simulink subsystem "Controller3w"  (R2025b)
settings: Solver=VariableStepAuto  StartTime=0.0  StopTime=10.0  RelTol=1e-3
undefined symbols (not defined in the file or in its folder): battery, controller, drivetrain
libraries: BatteryCurrentManagement x2
settings Model: Creator=jjha  LastModifiedBy=jjha
settings OptimizationCC: ReuseModelBlockBuffer=off
settings RTWCC: GPUComputeCapability=3.5

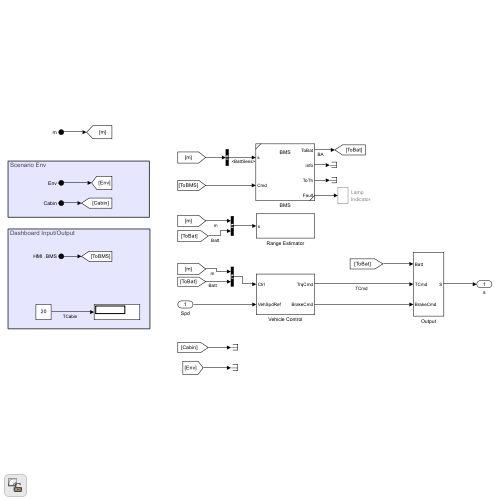
[thumbnail: Simulink's stored preview of the top-level diagram]
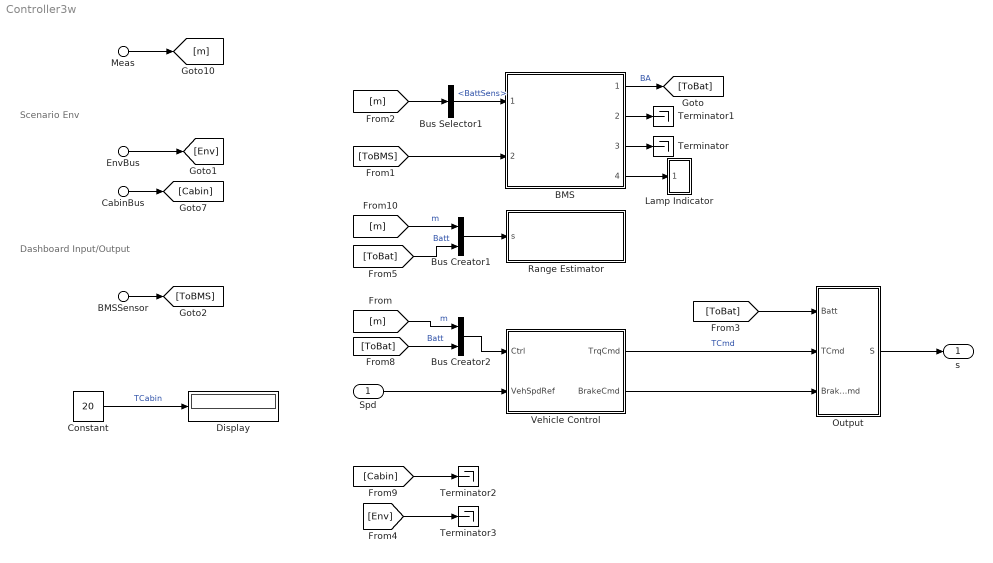
== system Controller3w ==
  note: Scenario Env
  note: Dashboard Input/Output
  Spd : Inport
  EnvBus : Inport  Port=2  PortName=Env
  CabinBus : Inport  Port=3  PortName=Cabin
  Meas : Inport  Port=4  PortName=m
  BMSSensor : Inport  Port=5  PortName=HMI  Element=BMS
  BMS : Subsystem  ReferencedSubsystem=BMS
      settings: PortSchema="{\"entries\":[{\"content\":{\"sides\":[{\"content\":{},\"type\":\"ConnectorPlacement.EquallySpacedRectSide\",\"uuid\":\"92c05094-f9b0-45a3-ac1b-1858c0c996e8\"},{\"content\":{\"side\":\"RIGHT\"},\"type\":\"ConnectorPlacement.EquallySpacedRectSide\",\"uuid\":\"cdc13757-7d0c-4e35-a976-de64c06d8cde\"},{\"content\":{\"connectorIds\":[\"In1\",\"In2\"],\"side\":\"TOP\"},\"type\":\"ConnectorPlacement.EquallySpacedRectSide\",\"uuid\":\"c53a1ad0-a5f6-468e-b5dd-f0a27cee9942\"},{\"content\":{\"connectorIds\":[\"Out1\",\"Out2\",\"Out3\",\"Out4\"],\"side\":\"BOTTOM\"},\"type\":\"ConnectorPlacement.EquallySpacedRectSide\",\"uuid\":\"8abfd502-0389-4393-bb18-f131709acb23\"}]},\"type\":\"ConnectorPlacement.EquallySpacedConnector\",\"uuid\":\"102d552e-f167-4796-a536-13938ac07fac\"}],\"packageUris\":[\"http://schema.mathworks.com/mf0/Connector/R2020b\"],\"version\":\"1.0\"}"
  Bus Creator1 : BusCreator  Inputs=2
  Bus Creator2 : BusCreator  Inputs=2
  Bus Selector1 : BusSelector  OutputSignals=BA.BattSens
  Constant : Constant  Value=20
  Display : Display
  Lamp Indicator : Subsystem
      settings: PortSchema="{\"entries\":[{\"content\":{\"sides\":[{\"content\":{\"connectorIds\":[]},\"type\":\"ConnectorPlacement.EquallySpacedRectSide\",\"uuid\":\"c55e4a0c-c727-4224-8aa6-2961c151763f\"},{\"content\":{\"connectorIds\":[],\"side\":\"RIGHT\"},\"type\":\"ConnectorPlacement.EquallySpacedRectSide\",\"uuid\":\"62aa4b95-0b95-454c-8041-b3e5f6582f45\"},{\"content\":{\"connectorIds\":[\"In1\"],\"side\":\"TOP\"},\"type\":\"ConnectorPlacement.EquallySpacedRectSide\",\"uuid\":\"0d235e8c-306c-4ade-b7e4-bd2fcf6610c8\"}]},\"type\":\"ConnectorPlacement.EquallySpacedConnector\",\"uuid\":\"6725a8d5-e875-410a-8026-694fde1b795b\"}],\"packageUris\":[\"http://schema.mathworks.com/mf0/Connector/R2020b\"],\"version\":\"1.0\"}"
  Output : Subsystem
  Range Estimator : Subsystem
  Terminator{,1..3} (4 alike) : Terminator
  Vehicle Control : Subsystem
  s : Outport
  wires:
  [ToBat] -> Bus Creator1/2  "Batt"
  Bus Selector1/1 -> BMS/1  "<BattSens>"
  BMS/2 -> Terminator1/1
  BMS/4 -> Lamp Indicator/1(" ")
  BMS/3 -> Terminator/1
  BMS/1 -> [ToBat]  "BA"
  Spd/1 -> Vehicle Control/2(VehSpdRef)
  Meas/1 -> [m]
  EnvBus/1 -> [Env]
  CabinBus/1 -> [Cabin]
  Bus Creator1/1 -> Range Estimator/1(s)
  [ToBat] -> Bus Creator2/2  "Batt"
  Bus Creator2/1 -> Vehicle Control/1(Ctrl)
  [m] -> Bus Creator2/1  "m"
  [m] -> Bus Selector1/1
  [m] -> Bus Creator1/1  "m"
  [ToBMS] -> BMS/2
  BMSSensor/1 -> [ToBMS]
  [Cabin] -> Terminator2/1
  Constant/1 -> Display/1  "TCabin"
  [Env] -> Terminator3/1
  Vehicle Control/2(BrakeCmd) -> Output/3(BrakeCmd)
  [ToBat] -> Output/1(Batt)
  Output/1(S) -> s/1
  Vehicle Control/1(TrqCmd) -> Output/2(TCmd)  "TCmd"

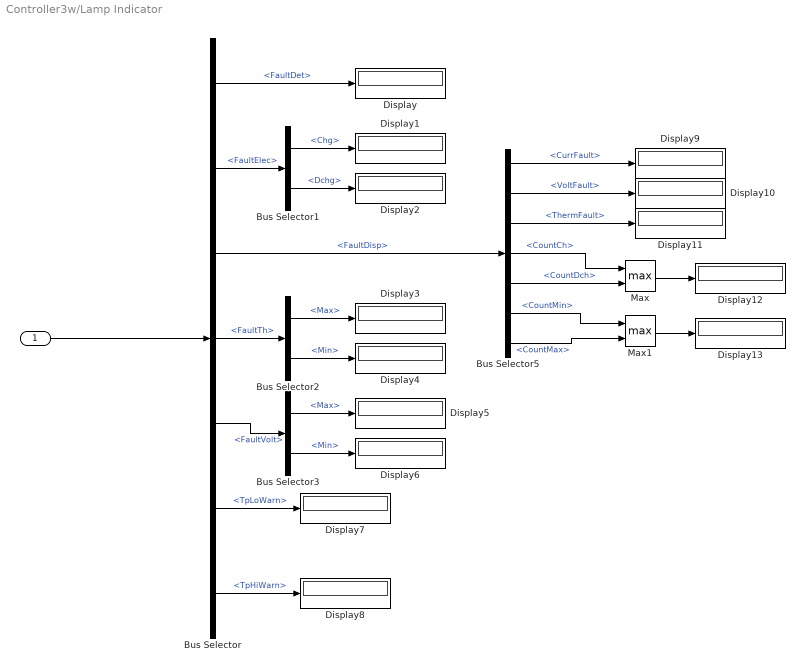
== system Controller3w/Lamp Indicator ==
  " " : Inport
  Bus Selector : BusSelector  OutputSignals=Fault.FaultDet,Fault.FaultElec,Fault.FaultDisp,Fault.FaultTh,Fault.FaultVolt,TpLoWarn,TpHiWarn
  Bus Selector1 : BusSelector  OutputSignals=Chg,Dchg
  Bus Selector2 : BusSelector  OutputSignals=Max,Min
  Bus Selector3 : BusSelector  OutputSignals=Max,Min
  Bus Selector5 : BusSelector  OutputSignals=CurrFault,VoltFault,ThermFault,CountCh,CountDch,CountMin,CountMax
  Display{,1..13} (14 alike) : Display
  Max : MinMax  Function=max  Inputs=2
  Max1 : MinMax  Function=max  Inputs=2
  wires:
  " "/1 -> Bus Selector/1
  Bus Selector/1 -> Display/1  "<FaultDet>"
  Bus Selector/2 -> Bus Selector1/1  "<FaultElec>"
  Bus Selector1/1 -> Display1/1  "<Chg>"
  Bus Selector1/2 -> Display2/1  "<Dchg>"
  Bus Selector/4 -> Bus Selector2/1  "<FaultTh>"
  Bus Selector2/2 -> Display4/1  "<Min>"
  Bus Selector2/1 -> Display3/1  "<Max>"
  Bus Selector3/1 -> Display5/1  "<Max>"
  Bus Selector3/2 -> Display6/1  "<Min>"
  Bus Selector/5 -> Bus Selector3/1  "<FaultVolt>"
  Bus Selector/6 -> Display7/1  "<TpLoWarn>"
  Bus Selector/7 -> Display8/1  "<TpHiWarn>"
  Bus Selector/3 -> Bus Selector5/1  "<FaultDisp>"
  Bus Selector5/1 -> Display9/1  "<CurrFault>"
  Bus Selector5/2 -> Display10/1  "<VoltFault>"
  Bus Selector5/3 -> Display11/1  "<ThermFault>"
  Bus Selector5/4 -> Max/1  "<CountCh>"
  Bus Selector5/6 -> Max1/1  "<CountMin>"
  Bus Selector5/7 -> Max1/2  "<CountMax>"
  Bus Selector5/5 -> Max/2  "<CountDch>"
  Max/1 -> Display12/1
  Max1/1 -> Display13/1

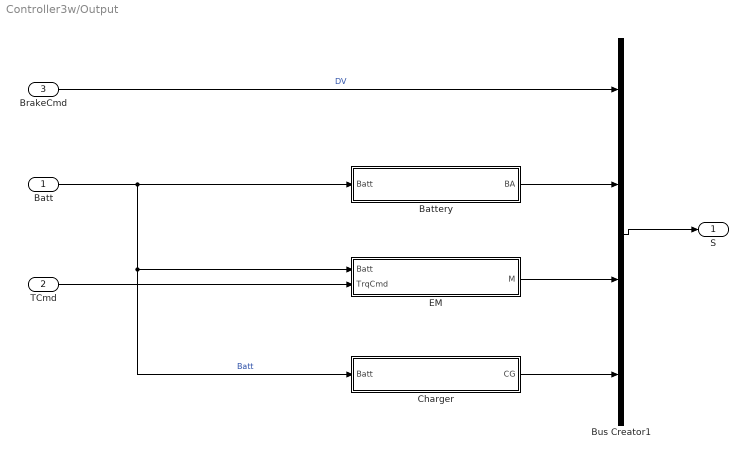
== system Controller3w/Output ==
  Batt : Inport
  TCmd : Inport  Port=2
  BrakeCmd : Inport  Port=3
  Battery : Subsystem
      mask Display: disp(get_param(gcb, 'Name'))
  Bus Creator1 : BusCreator  Inputs=4
  Charger : Subsystem
      mask Display: disp(get_param(gcb, 'Name'))
  EM : Subsystem
      mask Display: disp(get_param(gcb, 'Name'))
  S : Outport
  wires:
  Bus Creator1/1 -> S/1
  TCmd/1 -> EM/2(TrqCmd)
  EM/1(M) -> Bus Creator1/3
  Battery/1(BA) -> Bus Creator1/2
  Batt/1 -> Battery/1(Batt), EM/1(Batt), Charger/1(Batt)  "Batt"
  Charger/1(CG) -> Bus Creator1/4
  BrakeCmd/1 -> Bus Creator1/1  "DV"

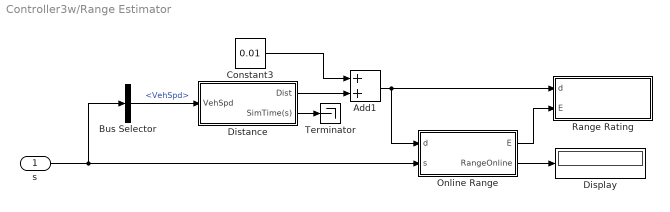
== system Controller3w/Range Estimator ==
  s : Inport
  Add1 : Sum
  Bus Selector : BusSelector  OutputSignals=m.DV.VehSpd
  Constant3 : Constant  Value=0.01
  Display : Display
  Distance : Subsystem
  Online Range : Subsystem
  Range Rating : Subsystem
  Terminator : Terminator
  wires:
  Online Range/1(E) -> Range Rating/2(E)
  Online Range/2(RangeOnline) -> Display/1
  s/1 -> Online Range/2(s), Bus Selector/1
  Constant3/1 -> Add1/1
  Bus Selector/1 -> Distance/1(VehSpd)  "<VehSpd>"
  Distance/2(SimTime(s)) -> Terminator/1
  Add1/1 -> Range Rating/1(d), Online Range/1(d)
  Distance/1(Dist) -> Add1/2

== system Controller3w/Vehicle Control ==
  Ctrl : Inport
  VehSpdRef : Inport  Port=2
  Bus Selector : BusSelector  OutputSignals=m.M.EM.EMrpm
  Driver : Subsystem
  Torque Control : Subsystem
  Torque Req : Subsystem
  TrqCmd : Outport
  BrakeCmd : Outport  Port=2
  wires:
  VehSpdRef/1 -> Driver/1(VehSpdRef)
  Bus Selector/1 -> Driver/2(rpm)  "<EMrpm>"
  Driver/1(TrqReq) -> Torque Control/1(TrqReq)
  Ctrl/1 -> Bus Selector/1, Torque Control/2(Crtl)
  Torque Req/1(TrqCmd) -> TrqCmd/1
  Torque Control/1(TrqCtrl) -> Torque Req/1(TrqCtrl)
  Torque Req/2(BrakeCmd) -> BrakeCmd/1

== system Controller3w/Output/Battery ==
  Batt : Inport
  Bus Creator : BusCreator  Inputs=2
  Bus Selector : BusSelector  OutputSignals=Relay.RelayPos,Relay.RelayNeg
  BA : Outport
  wires:
  Bus Selector/1 -> Bus Creator/1  "<RelayPos>"
  Batt/1 -> Bus Selector/1  "BA"
  Bus Selector/2 -> Bus Creator/2  "<RelayNeg>"
  Bus Creator/1 -> BA/1  "BA"

== system Controller3w/Output/Charger ==
  Batt : Inport
  Bus Creator : BusCreator  Inputs=1
  CG : Outport
  wires:
  Bus Creator/1 -> CG/1  "CG"
  Batt/1 -> Bus Creator/1  "Batt"

== system Controller3w/Output/EM ==
  Batt : Inport
  TrqCmd : Inport  Port=2
  Bus Creator3 : BusCreator  Inputs=2
  Bus Selector1 : BusSelector  OutputSignals=TorqueCmd
  Gain : Gain
  Scope : Scope
  M : Outport
  wires:
  Gain/1 -> Bus Creator3/1, Scope/1  "EMtrq"
  Batt/1 -> Bus Creator3/2
  Bus Creator3/1 -> M/1  "M"
  Bus Selector1/1 -> Gain/1  "<TorqueCmd>"
  TrqCmd/1 -> Bus Selector1/1

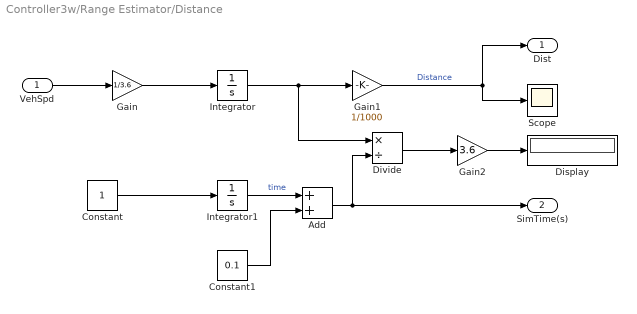
== system Controller3w/Range Estimator/Distance ==
  VehSpd : Inport
  Add : Sum
  Constant : Constant
  Constant1 : Constant  Value=0.1
  Display : Display
  Divide : Product  Inputs=*/
  Gain : Gain  Gain=1/3.6
  Gain1 : Gain  Gain=1/1000
  Gain2 : Gain  Gain=3.6
  Integrator : Integrator
  Integrator1 : Integrator
  Scope : Scope
      settings: ActiveDisplayYMinimum=-40.29184  ActiveDisplayYMaximum=362.62657  DataLoggingVariableName=ScopeData2
  Dist : Outport
  SimTime(s) : Outport  Port=2
  wires:
  Gain2/1 -> Display/1
  Gain1/1 -> Dist/1, Scope/1  "Distance"
  Gain/1 -> Integrator/1
  Divide/1 -> Gain2/1
  Add/1 -> SimTime(s)/1, Divide/2
  Integrator1/1 -> Add/1  "time"
  Constant1/1 -> Add/2
  Integrator/1 -> Divide/1, Gain1/1
  VehSpd/1 -> Gain/1
  Constant/1 -> Integrator1/1

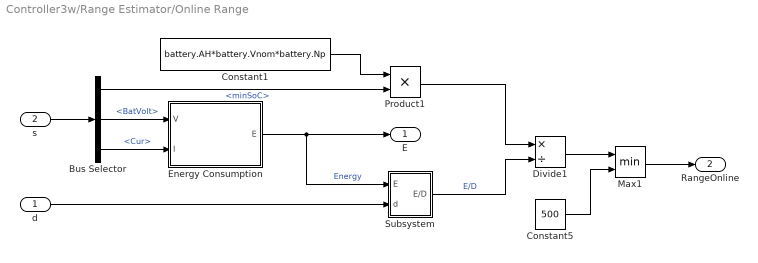
== system Controller3w/Range Estimator/Online Range ==
  d : Inport
  s : Inport  Port=2
  Bus Selector : BusSelector  OutputSignals=Batt.BattSensor.minSoC,Batt.BattSensor.BatVolt,Batt.BattSensor.Cur
  Constant1 : Constant  Value=battery.AH*battery.Vnom*battery.Np
  Constant5 : Constant  Value=500
  Divide1 : Product  Inputs=*/
  Energy Consumption : Subsystem
  Max1 : MinMax  Inputs=2  ZeroCross=off
  Product1 : Product
  Subsystem : Subsystem
  E : Outport
  RangeOnline : Outport  Port=2
  wires:
  Subsystem/1(E/D) -> Divide1/2  "E/D"
  d/1 -> Subsystem/2(d)
  Product1/1 -> Divide1/1
  Constant1/1 -> Product1/1
  Bus Selector/3 -> Energy Consumption/2(I)  "<Cur>"
  Bus Selector/2 -> Energy Consumption/1(V)  "<BatVolt>"
  Energy Consumption/1(E) -> E/1, Subsystem/1(E)  "Energy"
  s/1 -> Bus Selector/1
  Max1/1 -> RangeOnline/1
  Divide1/1 -> Max1/1
  Constant5/1 -> Max1/2
  Bus Selector/1 -> Product1/2  "<minSoC>"

== system Controller3w/Range Estimator/Range Rating ==
  note: Total capacity at full charge , Ahr*BatVoltage*CellinSeries
  d : Inport
  E : Inport  Port=2
  Add : Sum
  Constant : Constant
  Display : Display
  Divide : Product  Inputs=*/
  Divide1 : Product  Inputs=/*
  TotalEnergy : Constant  Value=battery.AH*battery.Vnom*battery.Np
  wires:
  Divide/1 -> Add/2
  Divide1/1 -> Display/1  "RangeRating"
  d/1 -> Divide/2
  E/1 -> Divide/1
  Constant/1 -> Add/1
  Add/1 -> Divide1/1
  TotalEnergy/1 -> Divide1/2

== system Controller3w/Vehicle Control/Driver ==
  VehSpdRef : Inport
  rpm : Inport  Port=2
  Motor Speed Reference : Subsystem
  Speed Controller : Subsystem
      settings: PortSchema="{\"entries\":[{\"content\":{\"sides\":[{\"content\":{\"connectorIds\":[\"Out1\"]},\"type\":\"ConnectorPlacement.EquallySpacedRectSide\",\"uuid\":\"12b9f2c9-2b28-451b-ad36-7fe4150db485\"},{\"content\":{\"connectorIds\":[\"In2\"],\"side\":\"RIGHT\"},\"type\":\"ConnectorPlacement.EquallySpacedRectSide\",\"uuid\":\"c0fdf9a4-483a-4ddc-b663-6299fcc79327\"},{\"content\":{\"connectorIds\":[\"In1\"],\"side\":\"TOP\"},\"type\":\"ConnectorPlacement.EquallySpacedRectSide\",\"uuid\":\"3f20082e-8487-45e3-9fd7-d6d75741df4d\"}]},\"type\":\"ConnectorPlacement.EquallySpacedConnector\",\"uuid\":\"9361cdd3-74d8-46ee-ae7f-e2dde5d31ed1\"}],\"packageUris\":[\"http://schema.mathworks.com/mf0/Connector/19700101\"],\"version\":\"1.0\"}"
  TrqReq : Outport
  wires:
  VehSpdRef/1 -> Motor Speed Reference/1(VehSpd)
  Speed Controller/1(TrqPID) -> TrqReq/1
  rpm/1 -> Speed Controller/1(Spd)
  Motor Speed Reference/1(MotorSpdRef) -> Speed Controller/2(SpdRef)

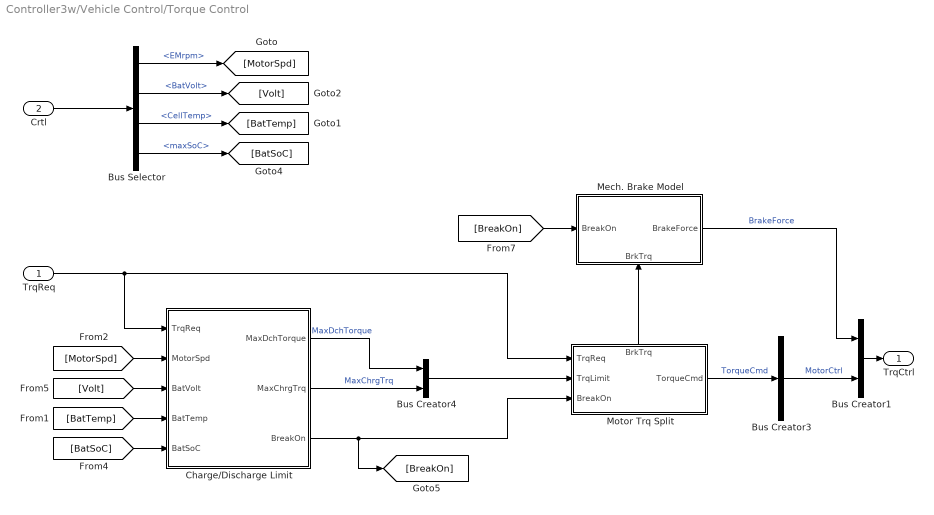
== system Controller3w/Vehicle Control/Torque Control ==
  TrqReq : Inport
  Crtl : Inport  Port=2
  Bus Creator1 : BusCreator  Inputs=2
  Bus Creator3 : BusCreator  Inputs=1
  Bus Creator4 : BusCreator  Inputs=2
  Bus Selector : BusSelector  OutputSignals=m.M.EM.EMrpm,Batt.BattSensor.BatVolt,Batt.BattSensor.CellTemp,Batt.BattSensor.maxSoC
  Charge/Discharge Limit : Subsystem
  Mech. Brake Model : Subsystem
      settings: PortSchema="{\"entries\":[{\"content\":{\"sides\":[{\"content\":{\"connectorIds\":[\"In1\"]},\"type\":\"ConnectorPlacement.EquallySpacedRectSide\",\"uuid\":\"3fcf8e06-a346-49b8-a4a8-b41cf2b27013\"},{\"content\":{\"connectorIds\":[\"Out1\"],\"side\":\"RIGHT\"},\"type\":\"ConnectorPlacement.EquallySpacedRectSide\",\"uuid\":\"8698242e-d004-4fda-889c-69f0784e7402\"},{\"content\":{\"connectorIds\":[],\"side\":\"TOP\"},\"type\":\"ConnectorPlacement.EquallySpacedRectSide\",\"uuid\":\"7829013b-7288-42bb-bccf-7e6edbe20d12\"},{\"content\":{\"connectorIds\":[\"In2\"],\"side\":\"BOTTOM\"},\"type\":\"ConnectorPlacement.EquallySpacedRectSide\",\"uuid\":\"357a4631-0a09-454f-b0f2-2b693ca62a9f\"},{\"content\":{\"connectorIds\":[],\"side\":\"HIDDEN\"},\"type\":\"ConnectorPlacement.EquallySpacedRectSide\",\"uuid\":\"b5eacf60-b578-4936-bef0-d59a279d5824\"}]},\"type\":\"ConnectorPlacement.EquallySpacedConnector\",\"uuid\":\"d2ebf12e-a3e7-4a55-b8c6-fa4e5ed13b89\"}],\"packageUris\":[\"http://schema.mathworks.com/mf0/Connector/R2020b\"],\"version\":\"1.0\"}"
  Motor Trq Split : Subsystem
      settings: PortSchema="{\"entries\":[{\"content\":{\"sides\":[{\"content\":{\"connectorIds\":[\"In1\",\"In2\",\"In3\"]},\"type\":\"ConnectorPlacement.EquallySpacedRectSide\",\"uuid\":\"c6883188-188e-4cbf-9dc5-1a26bf01b714\"},{\"content\":{\"connectorIds\":[\"Out1\"],\"side\":\"RIGHT\"},\"type\":\"ConnectorPlacement.EquallySpacedRectSide\",\"uuid\":\"b7c90991-838b-485d-9a4c-3fbacac28b54\"},{\"content\":{\"connectorIds\":[\"Out2\"],\"side\":\"TOP\"},\"type\":\"ConnectorPlacement.EquallySpacedRectSide\",\"uuid\":\"50e43671-3241-4bf5-a3b9-e23b27b7214a\"},{\"content\":{\"connectorIds\":[],\"side\":\"HIDDEN\"},\"type\":\"ConnectorPlacement.EquallySpacedRectSide\",\"uuid\":\"7c25a71e-e9cc-425c-8a3d-1b4aa412427f\"}]},\"type\":\"ConnectorPlacement.EquallySpacedConnector\",\"uuid\":\"d51dcaef-c892-4ef2-982d-c6c52760ceaa\"}],\"packageUris\":[\"http://schema.mathworks.com/mf0/Connector/R2020b\"],\"version\":\"1.0\"}"
  TrqCtrl : Outport
  wires:
  Crtl/1 -> Bus Selector/1
  Bus Selector/1 -> [MotorSpd]  "<EMrpm>"
  Bus Selector/4 -> [BatSoC]  "<maxSoC>"
  Bus Selector/2 -> [Volt]  "<BatVolt>"
  Bus Selector/3 -> [BatTemp]  "<CellTemp>"
  Charge/Discharge Limit/3(BreakOn) -> [BreakOn], Motor Trq Split/3(BreakOn)
  Charge/Discharge Limit/1(MaxDchTorque) -> Bus Creator4/1  "MaxDchTorque"
  TrqReq/1 -> Charge/Discharge Limit/1(TrqReq), Motor Trq Split/1(TrqReq)
  [MotorSpd] -> Charge/Discharge Limit/2(MotorSpd)
  [BatSoC] -> Charge/Discharge Limit/5(BatSoC)
  [BatTemp] -> Charge/Discharge Limit/4(BatTemp)
  [Volt] -> Charge/Discharge Limit/3(BatVolt)
  [BreakOn] -> Mech. Brake Model/1(BreakOn)
  Motor Trq Split/2(BrkTrq) -> Mech. Brake Model/2(BrkTrq)
  Charge/Discharge Limit/2(MaxChrgTrq) -> Bus Creator4/2  "MaxChrgTrq"
  Bus Creator4/1 -> Motor Trq Split/2(TrqLimit)
  Mech. Brake Model/1(BrakeForce) -> Bus Creator1/1  "BrakeForce"
  Bus Creator1/1 -> TrqCtrl/1
  Bus Creator3/1 -> Bus Creator1/2  "MotorCtrl"
  Motor Trq Split/1(TorqueCmd) -> Bus Creator3/1  "TorqueCmd"

== system Controller3w/Vehicle Control/Torque Req ==
  TrqCtrl : Inport
  Bus Selector1 : BusSelector  OutputSignals=BrakeForce,MotorCtrl.TorqueCmd
  TrqCmd : Outport
  BrakeCmd : Outport  Port=2
  wires:
  TrqCtrl/1 -> Bus Selector1/1
  Bus Selector1/2 -> TrqCmd/1  "<TorqueCmd>"
  Bus Selector1/1 -> BrakeCmd/1  "<BrakeForce>"

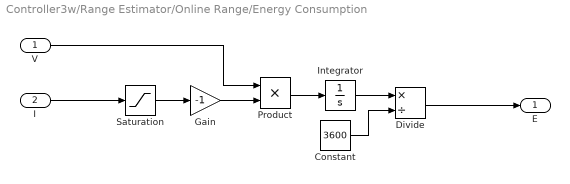
== system Controller3w/Range Estimator/Online Range/Energy Consumption ==
  V : Inport
  I : Inport  Port=2
  Constant : Constant  Value=3600
  Divide : Product  Inputs=*/
  Gain : Gain  Gain=-1
  Integrator : Integrator
  Product : Product
  Saturation : Saturate  UpperLimit=0  LowerLimit=-inf  ZeroCross=off
  E : Outport
  wires:
  Gain/1 -> Product/2
  Divide/1 -> E/1
  V/1 -> Product/1
  I/1 -> Saturation/1
  Product/1 -> Integrator/1
  Integrator/1 -> Divide/1
  Constant/1 -> Divide/2
  Saturation/1 -> Gain/1

== system Controller3w/Range Estimator/Online Range/Subsystem ==
  E : Inport
  d : Inport  Port=2
  Add : Sum
  Constant2 : Constant
  Divide2 : Product  Inputs=*/
  E/D : Outport
  wires:
  E/1 -> Divide2/1
  d/1 -> Divide2/2
  Divide2/1 -> Add/1
  Constant2/1 -> Add/2
  Add/1 -> E/D/1

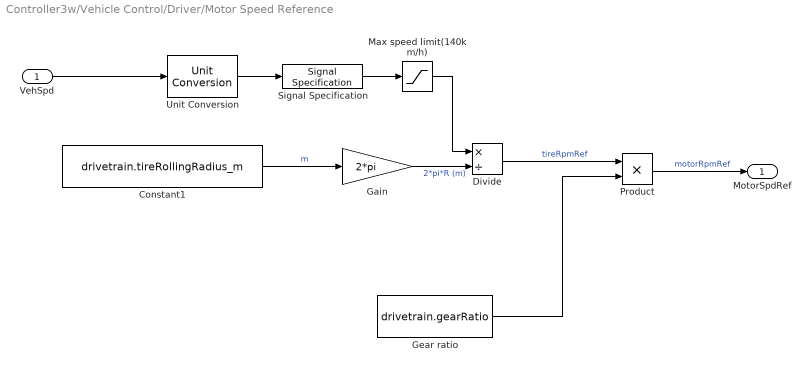
== system Controller3w/Vehicle Control/Driver/Motor Speed Reference ==
  VehSpd : Inport  Unit=km/hr
  Constant1 : Constant  Value=drivetrain.tireRollingRadius_m
  Divide : Product  Inputs=*/
  Gain : Gain  Gain=2*pi
  Gear ratio : Constant  Value=drivetrain.gearRatio
  Max speed limit(140km/h) : Saturate  UpperLimit=drivetrain.MaxSpeed  LowerLimit=0  ZeroCross=off
  Product : Product
  Signal Specification : SignalSpecification  Unit=m/min
  Unit Conversion : UnitConversion
  MotorSpdRef : Outport  Unit=rpm  VectorParamsAs1DForOutWhenUnconnected=off
  wires:
  Max speed limit(140km/h)/1 -> Divide/1
  VehSpd/1 -> Unit Conversion/1
  Product/1 -> MotorSpdRef/1  "motorRpmRef"
  Gear ratio/1 -> Product/2
  Divide/1 -> Product/1  "tireRpmRef"
  Gain/1 -> Divide/2  "2*pi*R (m)"
  Signal Specification/1 -> Max speed limit(140km/h)/1
  Unit Conversion/1 -> Signal Specification/1
  Constant1/1 -> Gain/1  "m"

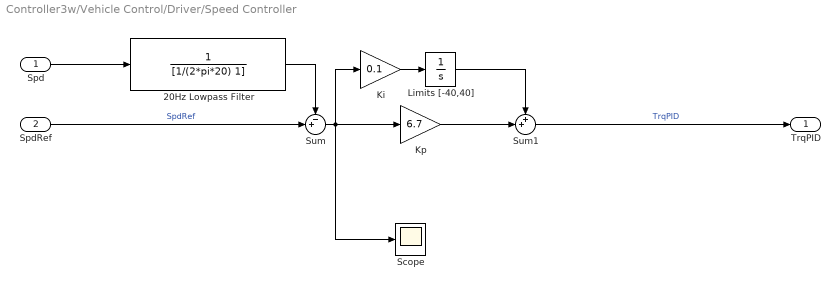
== system Controller3w/Vehicle Control/Driver/Speed Controller ==
  Spd : Inport  Unit=rpm
      settings: AttributesFormatString=%<Unit>
  SpdRef : Inport  Port=2  Unit=rpm
      settings: AttributesFormatString=%<Unit>
  20Hz Lowpass Filter : TransferFcn  Denominator=[1/(2*pi*20) 1]
  Ki : Gain  Gain=0.1
  Kp : Gain  Gain=6.7
  Limits [-40,40] : Integrator  LimitOutput=on  UpperSaturationLimit=40  LowerSaturationLimit=-40  ZeroCross=off
  Scope : Scope
      settings: ActiveDisplayYMinimum=-356.59933  ActiveDisplayYMaximum=2361.12393
  Sum : Sum  Inputs=-+|
  Sum1 : Sum  Inputs=++|
  TrqPID : Outport  Unit=N*m  VectorParamsAs1DForOutWhenUnconnected=off
      settings: AttributesFormatString=%<Unit>
  wires:
  SpdRef/1 -> Sum/2  "SpdRef"
  Spd/1 -> 20Hz Lowpass Filter/1
  Ki/1 -> Limits [-40,40]/1
  20Hz Lowpass Filter/1 -> Sum/1
  Sum/1 -> Ki/1, Kp/1, Scope/1
  Kp/1 -> Sum1/2
  Limits [-40,40]/1 -> Sum1/1
  Sum1/1 -> TrqPID/1  "TrqPID"

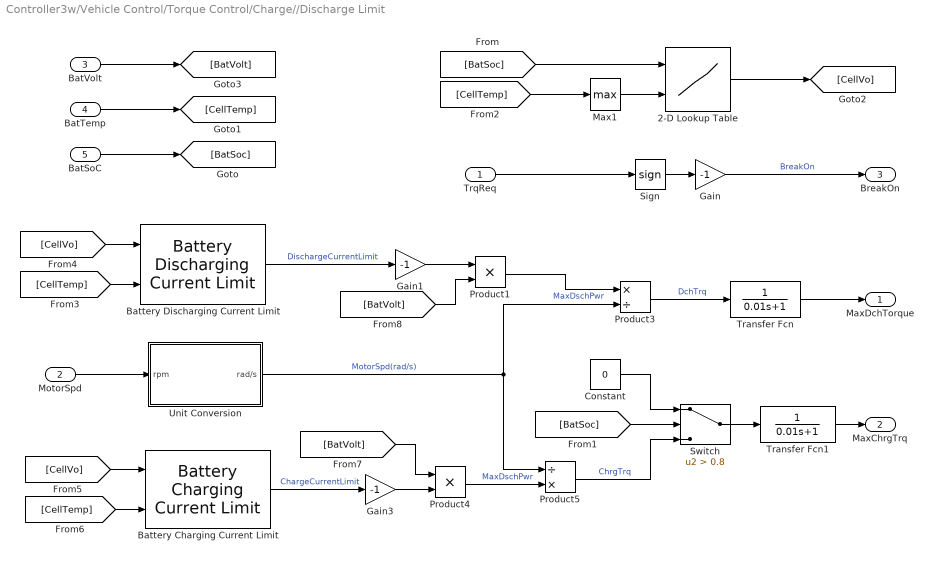
== system Controller3w/Vehicle Control/Torque Control/Charge//Discharge Limit ==
  TrqReq : Inport
  MotorSpd : Inport  Port=2
  BatVolt : Inport  Port=3
  BatTemp : Inport  Port=4
  BatSoC : Inport  Port=5
  2-D Lookup Table : Lookup_n-D  BreakpointsForDimension1=battery.SOC_vec  BreakpointsForDimension2=battery.T_vec  Table=battery.V0_mat  InternalRulePriority=Speed  RndMeth=Simplest
      settings: InputPortMap=u0,u1
  Battery Charging Current Limit : BatteryCurrentManagement/Battery Charging Current Limit  MinMaxFlag=off  CellOvervoltageLimit=4.5  R0=0.0025  T_vec=[243.15, 258.15, 273.15, 288.15, 303.15, 318.15, 333.15]  CurrentLimitCoolestCell=[ 0, 0,0.5* battery.AH, battery.AH, battery.AH, battery.AH, battery.AH]  CurrentLimitHottestCell="[ battery.AH,  battery.AH,  battery.AH,  battery.AH,  battery.AH,  0.5*battery.AH, 0]"  DataType=Inherit: auto
  Battery Discharging Current Limit : BatteryCurrentManagement/Battery Discharging Current Limit  MinMaxFlag=off  CellUndervoltageLimit=3  R0=0.0025  T_vec=[243.15, 258.15, 273.15, 288.15, 303.15, 318.15, 333.15]  CurrentLimitCoolestCell=[ 0, 0, battery.AH, battery.AH, battery.AH, battery.AH, battery.AH]  CurrentLimitHottestCell="[ 3*battery.AH,  3*battery.AH,  battery.AH,  battery.AH,  battery.AH,  battery.AH, 0]"  DataType=Inherit: auto
  Constant : Constant  Value=0
  Gain : Gain  Gain=-1
  Gain1 : Gain  Gain=-1
  Gain3 : Gain  Gain=-1
  Max1 : MinMax  Function=max  ZeroCross=off
  Product1 : Product
  Product3 : Product  Inputs=*/
  Product4 : Product
  Product5 : Product  Inputs=/*
  Sign : Signum  ZeroCross=off
  Switch : Switch  Criteria=u2 > Threshold  Threshold=0.8  SaturateOnIntegerOverflow=off  InputSameDT=off
  Transfer Fcn : TransferFcn  Denominator=[0.01 1]
  Transfer Fcn1 : TransferFcn  Denominator=[0.01 1]
  Unit Conversion : Subsystem
  MaxDchTorque : Outport
  MaxChrgTrq : Outport  Port=2
  BreakOn : Outport  Port=3
  wires:
  BatSoC/1 -> [BatSoc]
  Product1/1 -> Product3/1  "MaxDschPwr"
  Transfer Fcn1/1 -> MaxChrgTrq/1
  Constant/1 -> Switch/1
  [BatVolt] -> Product1/2
  BatVolt/1 -> [BatVolt]
  [CellTemp] -> Battery Charging Current Limit/2
  [CellVo] -> Battery Charging Current Limit/1
  2-D Lookup Table/1 -> [CellVo]
  [CellTemp] -> Max1/1
  BatTemp/1 -> [CellTemp]
  [BatSoc] -> Switch/2
  [BatSoc] -> 2-D Lookup Table/1
  [BatVolt] -> Product4/1
  Battery Discharging Current Limit/1 -> Gain1/1  "DischargeCurrentLimit"
  [CellVo] -> Battery Discharging Current Limit/1
  Max1/1 -> 2-D Lookup Table/2
  Switch/1 -> Transfer Fcn1/1
  Transfer Fcn/1 -> MaxDchTorque/1
  Gain1/1 -> Product1/1
  Product4/1 -> Product5/2  "MaxDschPwr"
  Gain3/1 -> Product4/2
  Battery Charging Current Limit/1 -> Gain3/1  "ChargeCurrentLimit"
  Product3/1 -> Transfer Fcn/1  "DchTrq"
  [CellTemp] -> Battery Discharging Current Limit/2
  MotorSpd/1 -> Unit Conversion/1(rpm)
  Unit Conversion/1(rad/s) -> Product5/1, Product3/2  "MotorSpd(rad/s)"
  Sign/1 -> Gain/1
  TrqReq/1 -> Sign/1
  Product5/1 -> Switch/3  "ChrgTrq"
  Gain/1 -> BreakOn/1  "BreakOn"

== system Controller3w/Vehicle Control/Torque Control/Mech. Brake Model ==
  BreakOn : Inport
  BrkTrq : Inport  Port=2
  Brake Force (N) : Constant  Value=0
  Switch : Switch  Criteria=u2 > Threshold  ZeroCross=off  SaturateOnIntegerOverflow=off  InputSameDT=off
  BrakeForce : Outport
  wires:
  BrkTrq/1 -> Switch/1
  Switch/1 -> BrakeForce/1
  Brake Force (N)/1 -> Switch/3
  BreakOn/1 -> Switch/2

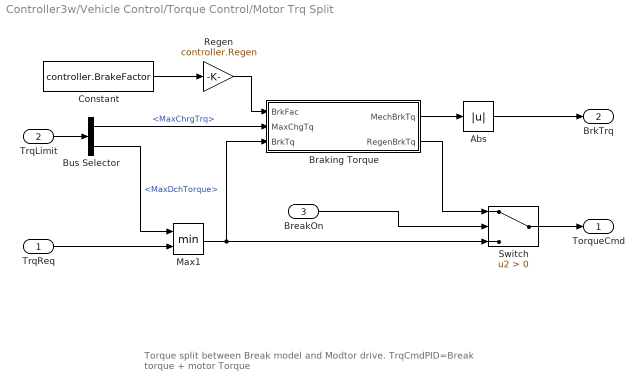
== system Controller3w/Vehicle Control/Torque Control/Motor Trq Split ==
  note: Torque split between Break model and Modtor drive.
      | TrqCmdPID=Break torque + motor Torque
  TrqReq : Inport
  TrqLimit : Inport  Port=2
  BreakOn : Inport  Port=3
  Abs : Abs  ZeroCross=off  SaturateOnIntegerOverflow=off
  Braking Torque : Subsystem
  Bus Selector : BusSelector  OutputSignals=MaxChrgTrq,MaxDchTorque
  Constant : Constant  Value=controller.BrakeFactor
  Max1 : MinMax  Inputs=2  ZeroCross=off
  Regen : Gain  Gain=controller.Regen
  Switch : Switch  Criteria=u2 > Threshold  ZeroCross=off  SaturateOnIntegerOverflow=off  InputSameDT=off
  TorqueCmd : Outport
  BrkTrq : Outport  Port=2
  wires:
  Regen/1 -> Braking Torque/1(BrkFac)
  Constant/1 -> Regen/1
  Bus Selector/1 -> Braking Torque/2(MaxChgTq)  "<MaxChrgTrq>"
  Abs/1 -> BrkTrq/1
  Braking Torque/1(MechBrkTq) -> Abs/1
  TrqLimit/1 -> Bus Selector/1
  Max1/1 -> Switch/3, Braking Torque/3(BrkTq)
  TrqReq/1 -> Max1/2
  Bus Selector/2 -> Max1/1  "<MaxDchTorque>"
  BreakOn/1 -> Switch/2
  Braking Torque/2(RegenBrkTq) -> Switch/1
  Switch/1 -> TorqueCmd/1

== system Controller3w/Vehicle Control/Torque Control/Charge//Discharge Limit/Unit Conversion ==
  rpm : Inport
  Add : Sum
  Constant : Constant
  Constant6 : Constant
  Product1 : Product
  Signal Specification : SignalSpecification  OutMin=[0]  Unit=rad/sec
  Unit Conversion : UnitConversion
  rad/s : Outport
  wires:
  Constant/1 -> Product1/1
  rpm/1 -> Unit Conversion/1
  Unit Conversion/1 -> Signal Specification/1
  Add/1 -> Product1/2
  Product1/1 -> rad/s/1
  Constant6/1 -> Add/2
  Signal Specification/1 -> Add/1

== system Controller3w/Vehicle Control/Torque Control/Motor Trq Split/Braking Torque ==
  BrkFac : Inport
  MaxChgTq : Inport  Port=2
  BrkTq : Inport  Port=3
  Add1 : Sum  Inputs=-+
  Max : MinMax  Function=max  Inputs=2  ZeroCross=off
  Product : Product
  MechBrkTq : Outport
  RegenBrkTq : Outport  Port=2
  wires:
  BrkFac/1 -> Product/1
  Product/1 -> Max/2
  BrkTq/1 -> Product/2, Add1/2
  Max/1 -> Add1/1, RegenBrkTq/1
  MaxChgTq/1 -> Max/1
  Add1/1 -> MechBrkTq/1
